simulink model "LunarMicrogrid_Combined_PVOnly"  (R2026b)
settings: Solver=ode23t  StopTime=simulation.timeSim  MaxStep=1/(5*solarPlant.converterSwitchingFrequency)  AbsTol=1e-3
PreLoadFcn:
  | run('LunarMicrogridA_Data');
undefined symbols (not defined in the file or in its folder): battery, bms, bmsController, connectedLoad, dcVoltage, lunarCase, maxSoC, maxVdc, minIrrad, minSoC, minVdc, olTime, sensor, solarPanel, solarPlant
libraries: fl_lib x14, nesl_utility x13, simulink x7, ee_lib x4, batteryecm_lib x1, simulink_extras x1, eePwmGenerator x1
(part 2 of 2)

== matlab function LunarMicrogrid_Combined_PVOnly/PV Converter ==
  data: G input; Ibus output; T input; Vbus input; en input; VmpT input; ImpT input; Pbus output; Pavail output; Vpv output; Ipv output; Imod output; duty output
function [Ibus, Pbus, Pavail, Vpv, Ipv, Imod, duty] = fcn(G,T,Vbus,en,VmpT,ImpT)
%#codegen
% EOL teammate MPP data; illustrative piecewise I-V fit.
% Shared PV bus, single coordinated P&O, six averaged PI branches.
persistent Vcmd dir Pprev count il integ
if isempty(Vcmd)
 Vcmd=217; dir=1; Pprev=0; count=0; il=zeros(6,1); integ=zeros(6,1);
end
dt=1e-4; eta=0.96; Gref=1367;
gs=max(0,min(1.5,G/Gref));
vmp=max(10,VmpT); imp=max(0,ImpT)*gs;
% Curve passes through Isc, Imp at Vmp, and zero at Voc.
% Isc=1.04 Imp, Voc=1.13 Vmp are MODEL ASSUMPTIONS.
isc=1.04*imp; voc=1.13*vmp;
Vcmd=max(0.5*vmp,min(0.99*voc,Vcmd));
if Vcmd<=vmp
 ipv=max(0,isc-(isc-imp)*(Vcmd/vmp)^2);
else
 ipv=max(0,imp*(voc-Vcmd)/(voc-vmp));
end
Ppv=Vcmd*ipv; Pavail=max(0,vmp*imp*eta);
count=count+1;
if count>=100
 if Ppv<Pprev, dir=-dir; end
 Vcmd=Vcmd+dir*0.5; Pprev=Ppv; count=0;
end
% Power-to-current reference; current limited by PV production.
v=max(30,Vbus);
Ptarget=max(0,min(Ppv*eta,Pavail))*max(0,min(1,en));
Iref=Ptarget/v/6;
Imod=zeros(6,1); duty=zeros(6,1);
for k=1:6
 % Averaged current PI with feedforward; shared-array duty proxy.
 err=Iref-il(k);
 dff=Vbus/max(1,1.15*Vcmd);
 d=max(0,min(0.85,dff+0.0015*err+integ(k)));
 % Average inductor dynamics; 33 uH each.
 next=il(k)+dt*(1.15*Vcmd*d-Vbus)/33e-6;
 % Avoid nonphysical reverse PV current.
 next=max(0,next);
 % Anti-windup: integrate only when unsaturated or correcting.
 if (d>0 && d<0.85) || (d<=0 && err>0) || (d>=0.85 && err<0)
  integ(k)=integ(k)+3*dt*err;
 end
 il(k)=next; Imod(k)=next; duty(k)=d;
end
% Conservation clamp: do not inject more power than PV can supply.
Iraw=sum(Imod); Ibus=min(Iraw,Ptarget/v);
Pbus=Ibus*max(0,Vbus); Vpv=Vcmd; Ipv=ipv;
end

== stateflow chart LunarMicrogrid_Combined_PVOnly/Mode Control ==
  state Mode2_BatCharge_pvMPPT
    entry:
    pvMPPT=1;
    BatCharge=1;
    modeNum=2;
    overload=0;
    exit:
    pvMPPT=0; BatCharge=0;
  state Start_Mode
    entry:
    ShutDown = 0;
    loadShutDown = 1;
    pvMPPT=0;
    VoltageControl=1;
    BatIsolate=1;
    modeNum=0;
    overload=0;
    exit:
    pvMPPT=0;
    BatIsolate=0;
    VoltageControl=0;
    loadShutDown = 0;
  state Mode5_System_ShutDown
    entry:
    PVoff=1; BatIsolate=1;
    ShutDown =1; modeNum=5;
    exit:
    ShutDown =0; PVoff=0;
    BatIsolate=0;
  state Mode1_batIsolated_pvVoltControl
    entry:
    VoltageControl=1; BatIsolate=1;
    modeNum=1;
    exit:
    VoltageControl=0; BatIsolate=0;
  state Mode6_pvMPPT_BatCharge_noload
    entry:
    pvMPPT=1; BatCharge=1;
    loadShutDown=1; modeNum=6;
    overload=1;
    exit:
    loadShutDown=0; pvMPPT=0;
    BatCharge=0;
  state Mode3_BatDischarge_pvMPPT
    entry:
    pvMPPT=1; BatDischarge=1;
    modeNum=3; overload=0;
    exit:
    pvMPPT=0;  BatDischarge=0;
  state Mode4_night_mode
    entry:
    PVoff=1; BatDischarge=1;
    modeNum=4;
    exit:
    PVoff=0; BatDischarge=0;
  Mode2_BatCharge_pvMPPT -> (junction 121) [order 3] : [Irrad<minIrrad && SoC>minSoC]
  Mode2_BatCharge_pvMPPT -> (junction 131) [order 2] : [Vdc < minVdc && SoC>minSoC]
  (junction 121) -> Mode4_night_mode
  (junction 131) -> (junction 154)
  Mode2_BatCharge_pvMPPT -> (junction 117) [order 5] : [Irrad<minIrrad && SoC<minSoC]
  (junction 132) -> Mode2_BatCharge_pvMPPT : [Vdc > maxVdc && Irrad>minIrrad]
  (junction 117) -> Mode5_System_ShutDown
  (junction 155) -> (junction 132)
  (junction 130) -> Mode2_BatCharge_pvMPPT : [(Irrad >minIrrad && overload==0) || ...
      | (overload==1 && rsflag==1)]
  Mode5_System_ShutDown -> (junction 130)
  Start_Mode -> Mode2_BatCharge_pvMPPT [order 1] : [SoC<minSoC]
  (junction 123) -> Mode2_BatCharge_pvMPPT
  Mode6_pvMPPT_BatCharge_noload -> (junction 123) [order 3] : [rsflag ==1 && Irrad > minIrrad  ...
      | && SoC <= minSoC]
  Mode2_BatCharge_pvMPPT -> (junction 125) [order 4]
  (default) -> Start_Mode
  (junction 125) -> Mode6_pvMPPT_BatCharge_noload : [duration(Vdc<minVdc)>olTime ...
      |  && SoC<minSoC]
  Mode2_BatCharge_pvMPPT -> Mode1_batIsolated_pvVoltControl [order 1] : [(SoC>maxSoC) || ...
      | (duration(Vdc>maxVdc)>olTime)]
  Start_Mode -> Mode3_BatDischarge_pvMPPT [order 2] : [SoC>minSoC]
  Mode1_batIsolated_pvVoltControl -> (junction 126)
  Mode6_pvMPPT_BatCharge_noload -> Mode5_System_ShutDown [order 2] : [(SoC<minSoC && ...
      | Irrad<minIrrad)|| ...
      | SoC>maxSoC]
  (junction 126) -> Mode3_BatDischarge_pvMPPT : [Vdc<minVdc]
  (junction 161) -> Mode5_System_ShutDown
  Mode4_night_mode -> Mode5_System_ShutDown [order 2] : [SoC<minSoC]
  Mode6_pvMPPT_BatCharge_noload -> (junction 127) [order 1] : [SoC>minSoC && rsflag==1]
  (junction 127) -> Mode3_BatDischarge_pvMPPT
  (junction 133) -> Mode6_pvMPPT_BatCharge_noload
  Mode3_BatDischarge_pvMPPT -> (junction 133) [order 2] : [(duration(Vdc<minVdc)>olTime || ...
      |  (SoC<minSoC && Vdc<minVdc)) && Irrad>minIrrad]
  Mode3_BatDischarge_pvMPPT -> (junction 161) [order 3] : [(SoC<minSoC && Irrad<minIrrad) || ( Irrad<minIrrad && duration(Vdc<minVdc)>olTime) ]
  Mode3_BatDischarge_pvMPPT -> (junction 155) [order 1]
  Mode4_night_mode -> Mode3_BatDischarge_pvMPPT [order 1] : [Irrad>minIrrad]
  Mode3_BatDischarge_pvMPPT -> Mode4_night_mode [order 4] : [Irrad<minIrrad && SoC>minSoC]
  (junction 154) -> Mode3_BatDischarge_pvMPPT
  data: Irrad input; Vdc input; SoC input; ShutDown output; maxSoC parameter; maxVdc parameter; minIrrad parameter; minSoC parameter; minVdc parameter; loadShutDown output; VoltageControl output; data output; BatCharge output; BatDischarge output; BatIsolate output; PVoff output; pvMPPT output; modeNum output; rsflag input; overload output; olTime parameter
